simulink model "my_tower"  (R2026b)
settings: Solver=ode1  StopTime=sim_days*86400  FixedStep=60
InitFcn:
  | tower_sim_init
values from neighbouring files (symbols this model uses):
  P_bat_Ah = cases{c,3}    [protection_test.m]
  P_Gmean = mean(cairo_w.G)    [tower_sim_init.m]
  P_panel_W = cases{c,2}    [protection_test.m]
  P_plants = p_.plants    [tower_sim_init.m]
  P_qpocket = min(tf_.pocket_Lph)    [tower_sim_init.m]
  P_Qtop = tf_.Q_Lph    [tower_sim_init.m]
  P_Vmax = p_.tank_usable_L    [tower_sim_init.m]
undefined symbols (not defined in the file or in its folder): P_autorefill
settings Model: Creator=HP  LastModifiedBy=HP

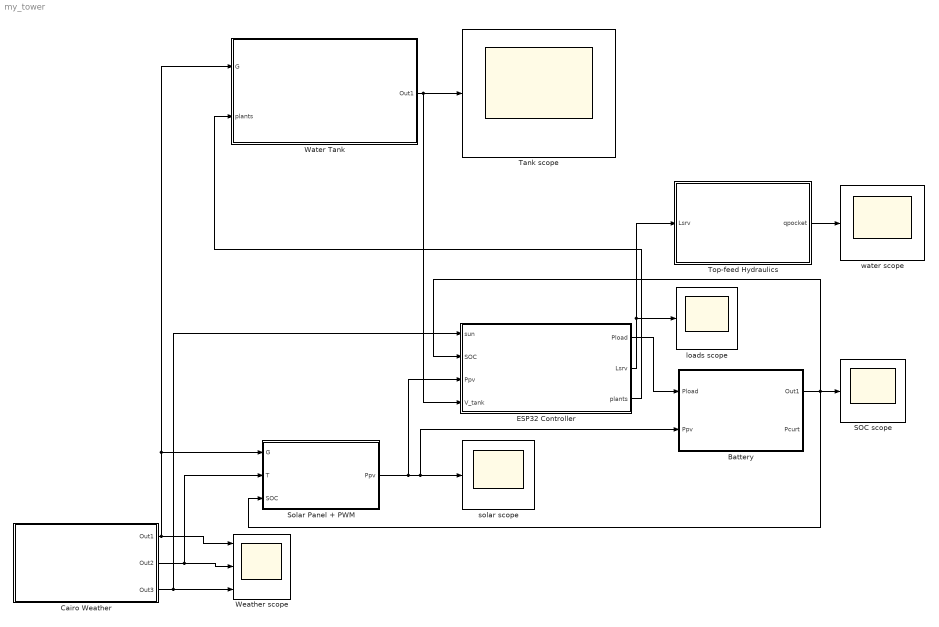
== system my_tower ==
  Battery : Subsystem
  Cairo Weather : Subsystem
  ESP32 Controller : Subsystem
  SOC scope : Scope
      settings: ActiveDisplayYMinimum=0.4470494859373923  ActiveDisplayYMaximum=0.95032783489584527  DataLoggingVariableName=ScopeData2
  Solar Panel + PWM : Subsystem
  Tank scope : Scope
      settings: ActiveDisplayYMinimum=1.7691363269002567  ActiveDisplayYMaximum=19.803429297011085  DataLoggingVariableName=ScopeData5
  Top-feed Hydraulics : Subsystem
  Water Tank : Subsystem
  "Weather scope " : Scope  NumInputPorts=3
      settings: ActiveDisplayYMinimum=-5.4856156825874178  ActiveDisplayYMaximum=13.250480321117463
  "loads scope " : Scope
      settings: ActiveDisplayYMinimum=-0.34730522819893994  ActiveDisplayYMaximum=5.0835960784779006  DataLoggingVariableName=ScopeData3
  "solar scope " : Scope
      settings: ActiveDisplayYMinimum=-4.7780561225977207  ActiveDisplayYMaximum=43.002505103379491
  "water scope " : Scope
      settings: ActiveDisplayYMinimum=-1.1049588048570127  ActiveDisplayYMaximum=9.9446292437131163  DataLoggingVariableName=ScopeData4
  wires:
  Cairo Weather/3(Out3) -> ESP32 Controller/1(sun), "Weather scope "/3
  Cairo Weather/2(Out2) -> "Weather scope "/2, Solar Panel + PWM/2(T)
  Cairo Weather/1(Out1) -> Solar Panel + PWM/1(G), Water Tank/1(G), "Weather scope "/1
  Water Tank/1(Out1) -> Tank scope/1, ESP32 Controller/4(V_tank)
  Solar Panel + PWM/1(Ppv) -> Battery/2(Ppv), "solar scope "/1, ESP32 Controller/3(Ppv)
  ESP32 Controller/3(plants) -> Water Tank/2(plants)
  ESP32 Controller/2(Lsrv) -> "loads scope "/1, Top-feed Hydraulics/1(Lsrv)
  ESP32 Controller/1(Pload) -> Battery/1(Pload)
  Top-feed Hydraulics/1(qpocket) -> "water scope "/1
  Battery/1(Out1) -> Solar Panel + PWM/3(SOC), ESP32 Controller/2(SOC), SOC scope/1

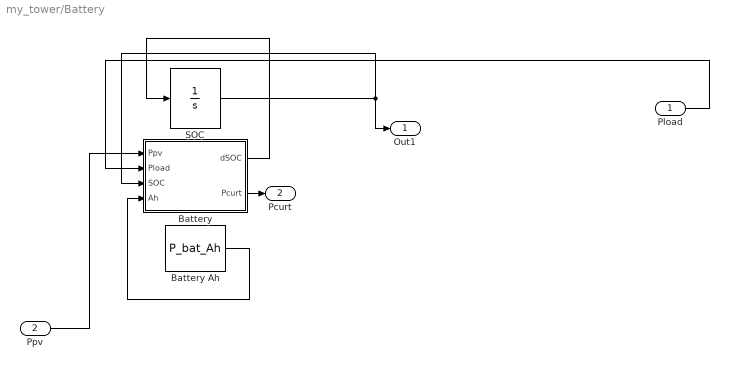
== system my_tower/Battery ==
  Pload : Inport
  Ppv : Inport  Port=2
  Battery : MATLAB Function  TreatAsAtomicUnit=on
  Battery Ah : Constant  Value=P_bat_Ah
  SOC : Integrator  InitialCondition=0.9  LimitOutput=on  UpperSaturationLimit=1  LowerSaturationLimit=0
  Out1 : Outport
  Pcurt : Outport  Port=2
  wires:
  Pload/1 -> Battery/2(Pload)
  Battery/1(dSOC) -> SOC/1
  SOC/1 -> Out1/1, Battery/3(SOC)
  Battery Ah/1 -> Battery/4(Ah)
  Battery/2(Pcurt) -> Pcurt/1
  Ppv/1 -> Battery/1(Ppv)

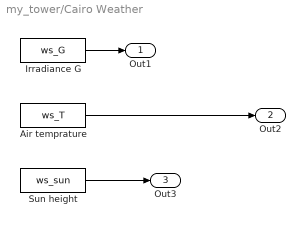
== system my_tower/Cairo Weather ==
  Air temprature : FromWorkspace  VariableName=ws_T  OutputAfterFinalValue=Holding final value
  Irradiance G : FromWorkspace  VariableName=ws_G  OutputAfterFinalValue=Holding final value
  Sun height : FromWorkspace  VariableName=ws_sun  OutputAfterFinalValue=Holding final value
  Out1 : Outport
  Out2 : Outport  Port=2
  Out3 : Outport  Port=3
  wires:
  Irradiance G/1 -> Out1/1
  Air temprature/1 -> Out2/1
  Sun height/1 -> Out3/1

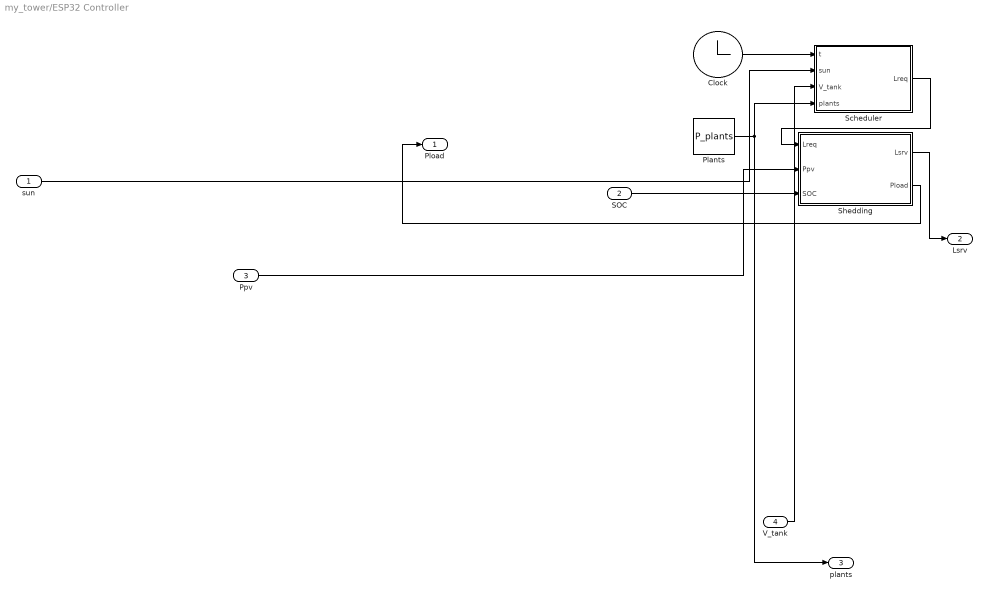
== system my_tower/ESP32 Controller ==
  sun : Inport
  SOC : Inport  Port=2
  Ppv : Inport  Port=3
  V_tank : Inport  Port=4
  Clock : Clock
  Plants : Constant  Value=P_plants
  Scheduler : MATLAB Function  TreatAsAtomicUnit=on
  Shedding : MATLAB Function  TreatAsAtomicUnit=on
  Pload : Outport
  Lsrv : Outport  Port=2
  plants : Outport  Port=3
  wires:
  Shedding/2(Pload) -> Pload/1
  Clock/1 -> Scheduler/1(t)
  V_tank/1 -> Scheduler/3(V_tank)
  sun/1 -> Scheduler/2(sun)
  Ppv/1 -> Shedding/2(Ppv)
  SOC/1 -> Shedding/3(SOC)
  Scheduler/1(Lreq) -> Shedding/1(Lreq)
  Plants/1 -> plants/1, Scheduler/4(plants)
  Shedding/1(Lsrv) -> Lsrv/1

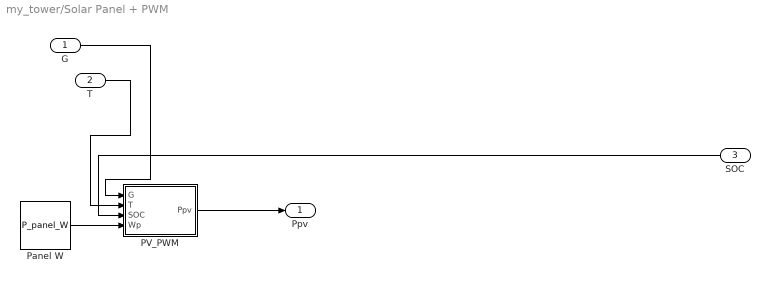
== system my_tower/Solar Panel + PWM ==
  G : Inport
  T : Inport  Port=2
  SOC : Inport  Port=3
  PV_PWM : MATLAB Function  TreatAsAtomicUnit=on
  Panel W : Constant  Value=P_panel_W
  Ppv : Outport
  wires:
  SOC/1 -> PV_PWM/3(SOC)
  Panel W/1 -> PV_PWM/4(Wp)
  PV_PWM/1(Ppv) -> Ppv/1
  G/1 -> PV_PWM/1(G)
  T/1 -> PV_PWM/2(T)

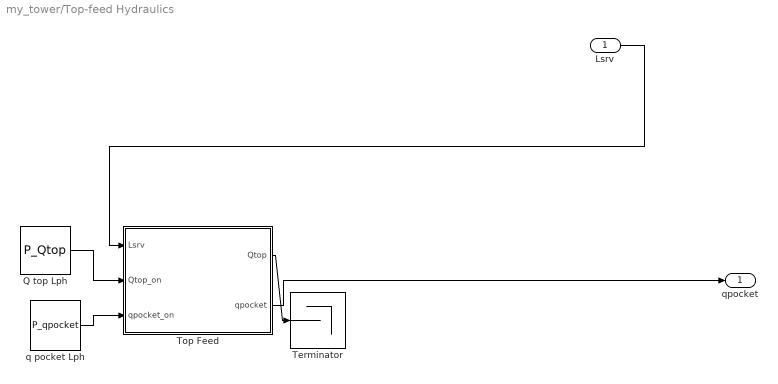
== system my_tower/Top-feed Hydraulics ==
  Lsrv : Inport
  Q top Lph : Constant  Value=P_Qtop
  Terminator : Terminator
  Top Feed : MATLAB Function  TreatAsAtomicUnit=on
  q pocket Lph : Constant  Value=P_qpocket
  qpocket : Outport
  wires:
  Top Feed/1(Qtop) -> Terminator/1
  Q top Lph/1 -> Top Feed/2(Qtop_on)
  Lsrv/1 -> Top Feed/1(Lsrv)
  Top Feed/2(qpocket) -> qpocket/1
  q pocket Lph/1 -> Top Feed/3(qpocket_on)

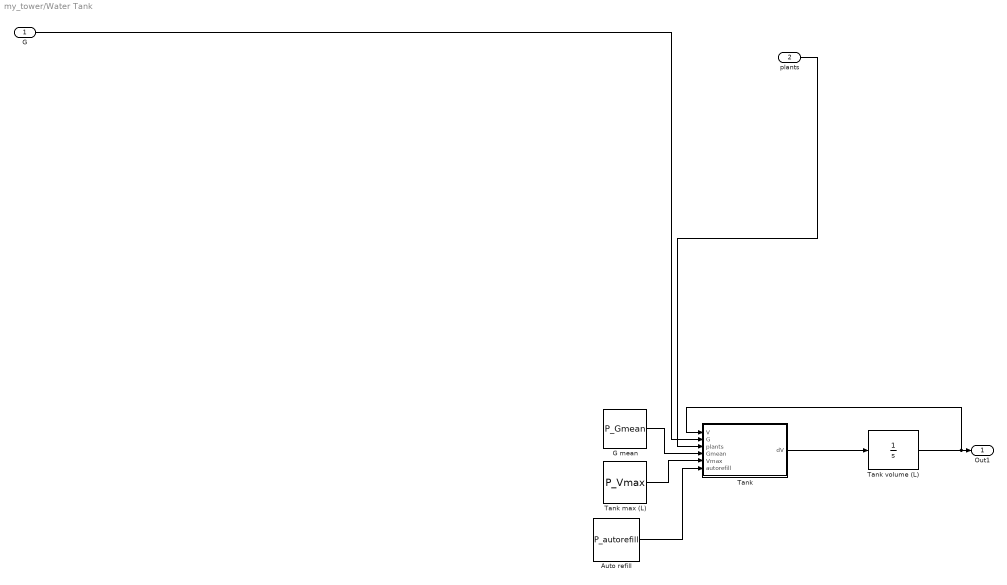
== system my_tower/Water Tank ==
  G : Inport
  plants : Inport  Port=2
  Auto refill : Constant  Value=P_autorefill
  G mean : Constant  Value=P_Gmean
  Tank : MATLAB Function  TreatAsAtomicUnit=on
  Tank max (L) : Constant  Value=P_Vmax
  Tank volume (L) : Integrator  InitialCondition=P_Vmax  LimitOutput=on  UpperSaturationLimit=P_Vmax  LowerSaturationLimit=0
  Out1 : Outport
  wires:
  G mean/1 -> Tank/4(Gmean)
  G/1 -> Tank/2(G)
  Tank/1(dV) -> Tank volume (L)/1
  plants/1 -> Tank/3(plants)
  Tank max (L)/1 -> Tank/5(Vmax)
  Tank volume (L)/1 -> Tank/1(V), Out1/1
  Auto refill/1 -> Tank/6(autorefill)

== matlab function my_tower/Battery/Battery ==
  data: Ppv input; dSOC output; Pload input; SOC input; Ah input; Pcurt output
function [dSOC, Pcurt] = Battery(Ppv, Pload, SOC, Ah)
% Lead-acid: 85 % charge eff., 97 % discharge eff., 0.25C limit, taper above 85 %
Cwh = 12*Ah;  net = Ppv - Pload;  Pcurt = 0;
if net >= 0
    acc = 0.25*Ah*12;                              % max charge power
    if SOC > 0.85, acc = acc*(1 - SOC)/0.15; end   % slows down when nearly full
    chg = min(net, acc);  dSOC = chg*0.85/Cwh/3600;  Pcurt = net - chg;
else
    dSOC = net/0.97/Cwh/3600;
end

== matlab function my_tower/Solar Panel + PWM/PV_PWM ==
  data: G input; Ppv output; T input; SOC input; Wp input
function Ppv = PV_PWM(G, T, SOC, Wp)
% 18 V panel + PWM controller: panel current at battery voltage
Tc  = T + G*25/800;              % cell temperature (NOCT 45 C)
Vb  = 11.9 + (14.2 - 11.9)*SOC;  % lead-acid voltage while charging
Imp = Wp/18;                     % panel current at max power
Ppv = max(0, Vb*Imp*1.08*G/1000*(1 + 0.0005*(Tc - 25))*0.90);  % 0.90 dust/wiring

== matlab function my_tower/ESP32 Controller/Scheduler ==
  data: t input; Lreq output; sun input; V_tank input; plants input
function Lreq = Scheduler(t, sun, V_tank, plants)
% ESP32 timetable. Lreq = requested power [ESP32 main air dosing Jetson] (W)
hr  = mod(t/3600, 24);  mn = mod(t/60, 60);  day = sun > 0;
if day
    pump = mn < 15;               air = mn >= 20 && mn < 35;   % 15 min/h
else
    pump = mod(floor(hr),2) == 0 && mn < 5;  air = mn >= 20 && mn < 26;  % night eco mode
end
pump = pump && V_tank > 0.5;      % float switch: never run the pump dry
dose = hr >= 10 && hr < 10 + 0.05*plants/60;
tc = [8 9.5 11 12.5 14 15.5];  tchk = (1.5 + 0.5*plants/8)/60;  jet = false;
for k = 1:numel(tc)
    if hr >= tc(k) && hr < tc(k) + tchk && sun >= 15, jet = true; end
end
Lreq = [0.8; 19.36*double(pump); 5.36*double(air); 5.36*double(dose); 12.56*double(jet)];

== matlab function my_tower/ESP32 Controller/Shedding ==
  data: Lreq input; Lsrv output; Ppv input; SOC input; Pload output
function [Lsrv, Pload] = Shedding(Lreq, Ppv, SOC)
% ESP32 battery protection: at minimum SOC, switch off loads in priority
% order Jetson -> air pump -> dosing -> main pump -> ESP32 until solar covers them.
Lsrv = Lreq;  order = [5 3 4 2 1];
if SOC <= 0.502
    for k = 1:5
        if sum(Lsrv) <= Ppv, break; end
        i = order(k);  Lsrv(i) = max(0, Lsrv(i) - (sum(Lsrv) - Ppv));
    end
end
Pload = sum(Lsrv);

== matlab function my_tower/Top-feed Hydraulics/Top Feed ==
  data: Lsrv input; Qtop output; Qtop_on input; qpocket_on input; qpocket output
function [Qtop, qpocket] = TopFeed(Lsrv, Qtop_on, qpocket_on)
% Pump lifts water to the top; drip trays feed 8 pockets per module.
% Operating point (from topfeed.m) scaled by the share of pump power served.
on = Lsrv(2)/19.36;
Qtop = Qtop_on*on;  qpocket = qpocket_on*on;

== matlab function my_tower/Water Tank/Tank ==
  settings: updateMethod=DISCRETE  sampleTime=60
  data: V input; dV output; G input; plants input; Gmean input; Vmax input; autorefill input
function dV = Tank(V, G, plants, Gmean, Vmax, autorefill)
% Water balance: plants drink 0.35 L/plant/day (scaled with sunshine);
% optional refill valve opens below 20 % and closes when full (10 L/min).
persistent refilling
if isempty(refilling), refilling = false; end
if autorefill > 0
    if V < 0.2*Vmax, refilling = true; end
    if V >= Vmax,    refilling = false; end
end
dV = -plants*0.35/86400*G/max(Gmean, 1) + double(refilling)*10/60;
